simulink model "gauss_markov"  (Simulink 4.00)
settings: Solver=ode45  StartTime=0.0  StopTime=10.0  RelTol=1e-3
values from neighbouring files (symbols this model uses):
  a = 6378137.0    (= 6378137)    [ecef2geo.m]
  b = 6356752.3142    [ecef2geo.m]
libraries: simulink3 x2
settings Model: Creator=mcar  LastModifiedBy=mcar  BlockReductionOpt=off

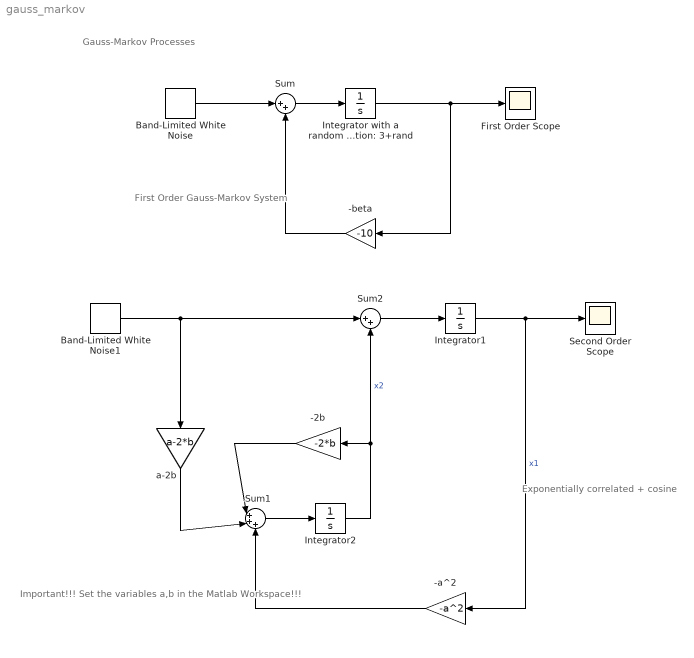
== system gauss_markov ==
  note: Gauss-Markov Processes
  note: Important!!!
      | Set the variables a,b in the
      | Matlab Workspace!!!
  note: First Order
      | Gauss-Markov System
  note: Exponentially correlated +
      | cosine
  -2b : Gain  Orientation=left  Gain=-2*b  Multiplication=Element-wise(K.*u)  SaturateOnIntegerOverflow=on
  -a^2 : Gain  Orientation=left  Gain=-a^2  Multiplication=Element-wise(K.*u)  SaturateOnIntegerOverflow=on
  -beta : Gain  Orientation=left  Gain=-10  Multiplication=Element-wise(K.*u)  SaturateOnIntegerOverflow=on
  Band-Limited White Noise : simulink3/Sources/Band-Limited White Noise  Cov=[10]  Ts=0.01  seed=[23341]
  Band-Limited White Noise1 : simulink3/Sources/Band-Limited White Noise  Cov=[10]  Ts=0.01  seed=[23341]
  First Order Scope : Scope
      settings: TimeRange=10  YMin=2  YMax=4.5  SaveToWorkspace=off  SaveName=ScopeData  LimitDataPoints=on  MaxDataPoints=5000
  Integrator with a random initial condition: 3+rand : Integrator  ExternalReset=none  InitialConditionSource=internal  InitialCondition=0  LimitOutput=off  UpperSaturationLimit=inf  LowerSaturationLimit=-inf  ShowSaturationPort=off  ShowStatePort=off  AbsoluteTolerance=auto
  Integrator1 : Integrator  ExternalReset=none  InitialConditionSource=internal  InitialCondition=0  LimitOutput=off  UpperSaturationLimit=inf  LowerSaturationLimit=-inf  ShowSaturationPort=off  ShowStatePort=off  AbsoluteTolerance=auto
  Integrator2 : Integrator  ExternalReset=none  InitialConditionSource=internal  InitialCondition=0  LimitOutput=off  UpperSaturationLimit=inf  LowerSaturationLimit=-inf  ShowSaturationPort=off  ShowStatePort=off  AbsoluteTolerance=auto
  Second Order Scope : Scope
      settings: TimeRange=10  YMin=2  YMax=4.5  SaveToWorkspace=off  LimitDataPoints=on  MaxDataPoints=5000
  Sum : Sum  Inputs=|++  SaturateOnIntegerOverflow=on
  Sum1 : Sum  Inputs=|+++  SaturateOnIntegerOverflow=on
  Sum2 : Sum  Inputs=|++  SaturateOnIntegerOverflow=on
  a-2b : Gain  Orientation=down  Gain=a-2*b  Multiplication=Element-wise(K.*u)  SaturateOnIntegerOverflow=on
  wires:
  Integrator with a random initial condition: 3+rand/1 -> -beta/1, First Order Scope/1
  -beta/1 -> Sum/2
  Sum/1 -> Integrator with a random initial condition: 3+rand/1
  Band-Limited White Noise/1 -> Sum/1
  Integrator1/1 -> Second Order Scope/1, -a^2/1  "x1"
  Band-Limited White Noise1/1 -> Sum2/1, a-2b/1
  Integrator2/1 -> -2b/1, Sum2/2  "x2"
  -2b/1 -> Sum1/1
  a-2b/1 -> Sum1/2
  Sum1/1 -> Integrator2/1
  -a^2/1 -> Sum1/3
  Sum2/1 -> Integrator1/1
